simulink model "Comunicacion_arduino_serial_obsevador_Fran"  (R2026a)
settings: Solver=VariableStepAuto  StopTime=100
libraries: instrumentseriallib x3, simulink x1
settings Model: Creator=Claudio  LastModifiedBy=CuadradoGris
settings DebuggingCC: UnderspecifiedInitializationDetection=Classic

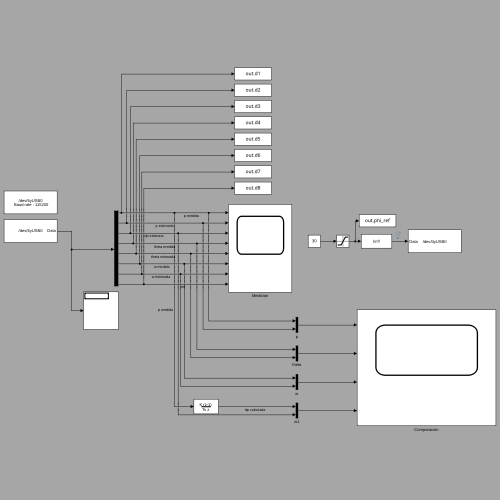
[thumbnail: Simulink's stored preview of the top-level diagram]
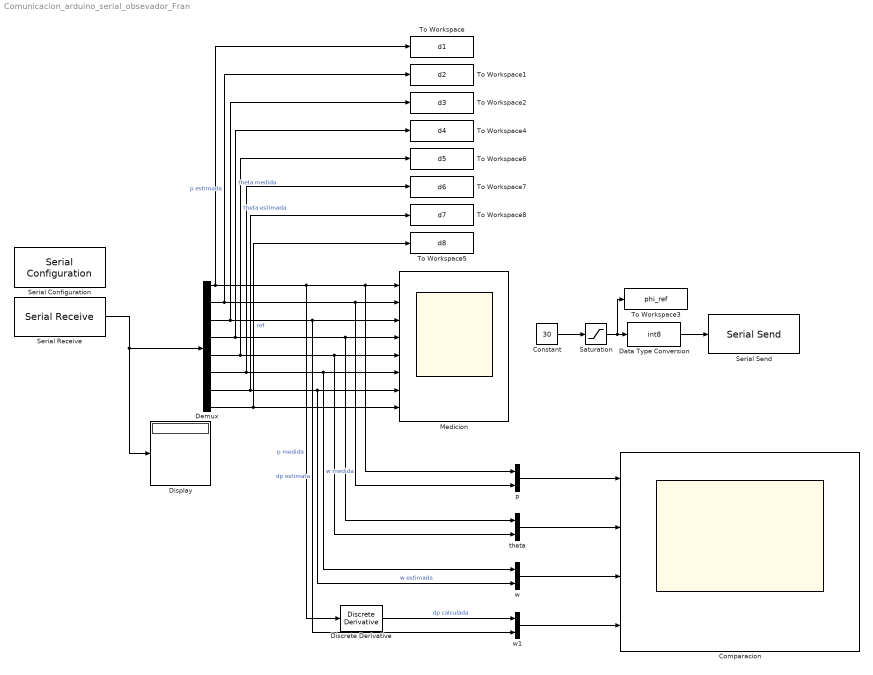
== system Comunicacion_arduino_serial_obsevador_Fran ==
  Comparacion : Scope  NumInputPorts=4
      settings: ActiveDisplayYMinimum=-1  ActiveDisplayYMaximum=1  DataLoggingSaveFormat=Array
  Constant : Constant  Value=30
  Data Type Conversion : DataTypeConversion  OutDataTypeStr=int8  SaturateOnIntegerOverflow=off  RndMeth=Floor
  Demux : Demux  Outputs=8
  Discrete Derivative : simulink/Discrete/Discrete Derivative  gainval=1.0  ICPrevScaledInput=0.0  OutMin=[]  OutMax=[]  OutDataType=fixdt(1, 16)  OutScaling=2^-10  DoSatur=off
  Display : Display
  Medicion : Scope  NumInputPorts=8
      settings: TimeSpan=100  ActiveDisplayYMinimum=-10.169571399688721  ActiveDisplayYMaximum=10.402695178985596  DataLoggingSaveFormat=Array
  Saturation : Saturate  UpperLimit=45  LowerLimit=-45
  Serial Configuration : instrumentseriallib/Serial Configuration  Priority=-200000  PortSel=/dev/ttyUSB0  Port=/dev/ttyUSB0  ComPort=/dev/ttyUSB0  BaudRate=115200  DataBits=8  Parity=none  StopBits=1  ByteOrder=little-endian  FlowControl=none  Timeout=10  SimulateUsing=Interpreted execution  BlockInModel=on  aMode=1
  Serial Receive : instrumentseriallib/Serial Receive  Priority=1  PortSel=/dev/ttyUSB0  Port=/dev/ttyUSB0  ComPort=/dev/ttyUSB0  DataType=single  SaveDataType=uint8  ToggleHeader=on  Header="[ 97   98   99  100 ]"  ToggleDataSize=on  DataSize=[8 1]  ToggleTerminator=off  Terminator=<none>  CustomTerminator=[]  InputFormat=Column major  EnableBlockingMode=on  ActionDataUnavailable=Output last received value  ActionWhenDataUnavailable=Output last received value  CustomValue=0  SampleTime=0.02  SimulateUsing=Interpreted execution  BlockInModel=on  aMode=1  LibraryInUse=instrumentlib
  Serial Send : instrumentseriallib/Serial Send  Priority=1  PortSel=/dev/ttyUSB0  Port=/dev/ttyUSB0  ComPort=/dev/ttyUSB0  Header=[]  Terminator=<none>  CustomTerminator=[]  EnableBlockingMode=on  SimulateUsing=Interpreted execution  BlockInModel=on  aMode=1
  To Workspace : ToWorkspace  VariableName=d1  SampleTime=-1
      settings: Save2DSignal=2-D array (concatenate along first dimension)
  To Workspace1 : ToWorkspace  VariableName=d2  SampleTime=-1
      settings: Save2DSignal=2-D array (concatenate along first dimension)
  To Workspace2 : ToWorkspace  VariableName=d3  SampleTime=-1
      settings: Save2DSignal=2-D array (concatenate along first dimension)
  To Workspace3 : ToWorkspace  VariableName=phi_ref  SampleTime=0.02
      settings: Save2DSignal=2-D array (concatenate along first dimension)
  To Workspace4 : ToWorkspace  VariableName=d4  SampleTime=-1
      settings: Save2DSignal=2-D array (concatenate along first dimension)
  To Workspace5 : ToWorkspace  VariableName=d8  SampleTime=-1
      settings: Save2DSignal=2-D array (concatenate along first dimension)
  To Workspace6 : ToWorkspace  VariableName=d5  SampleTime=-1
      settings: Save2DSignal=2-D array (concatenate along first dimension)
  To Workspace7 : ToWorkspace  VariableName=d6  SampleTime=-1
      settings: Save2DSignal=2-D array (concatenate along first dimension)
  To Workspace8 : ToWorkspace  VariableName=d7  SampleTime=-1
      settings: Save2DSignal=2-D array (concatenate along first dimension)
  p : Mux  Inputs=2
  theta : Mux  Inputs=2
  w : Mux  Inputs=2
  w1 : Mux  Inputs=2
  wires:
  Demux/2 -> p/2, Medicion/2, To Workspace1/1  "p estimada"
  Demux/1 -> Discrete Derivative/1, p/1, Medicion/1, To Workspace/1  "p medida"
  Demux/3 -> w1/2, Medicion/3, To Workspace2/1  "dp estimata"
  Constant/1 -> Saturation/1
  Saturation/1 -> To Workspace3/1, Data Type Conversion/1
  Demux/4 -> To Workspace4/1, theta/1, Medicion/4  "theta medida"
  p/1 -> Comparacion/1
  Serial Receive/1 -> Display/1, Demux/1
  Data Type Conversion/1 -> Serial Send/1
  Demux/5 -> To Workspace6/1, theta/2, Medicion/5  "theta estimada"
  Demux/8 -> To Workspace5/1, Medicion/8  "ref"
  Demux/6 -> To Workspace7/1, w/1, Medicion/6  "w medida"
  Demux/7 -> To Workspace8/1, w/2, Medicion/7  "w estimada"
  w/1 -> Comparacion/3
  theta/1 -> Comparacion/2
  w1/1 -> Comparacion/4
  Discrete Derivative/1 -> w1/1  "dp calculada"
